simulink model "motor_dc_machine_block"  (R2025a)
settings: Solver=VariableStepAuto  StartTime=0.0  StopTime=2  RelTol=1e-3
undefined symbols (not defined in the file): J_m, kfi, L_a, R_a, T_n, V_an
libraries: spsControlledVoltageSourceLib x1, spsDCMachineLib x1, sps_lib x1
settings Model: Creator=SCH 2  LastModifiedBy=SCH 2

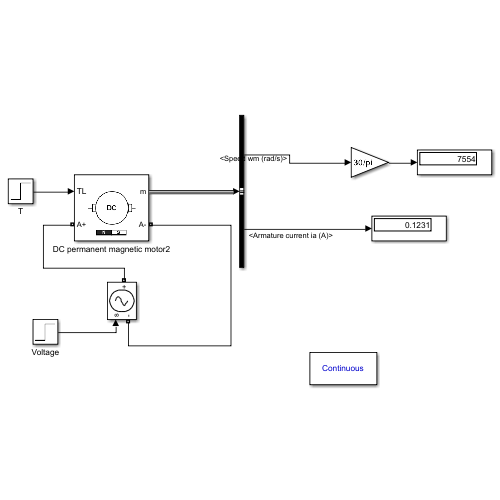
[thumbnail: Simulink's stored preview of the top-level diagram]
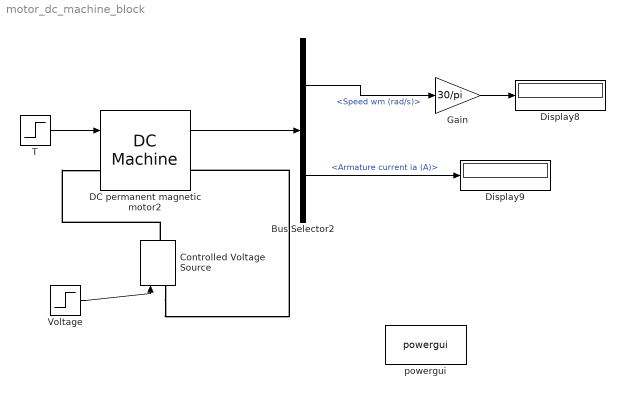
== system motor_dc_machine_block ==
  Bus Selector2 : BusSelector  OutputSignals=Speed wm (rad/s),Armature current ia (A)
  Controlled Voltage Source : spsControlledVoltageSourceLib/Controlled Voltage Source  Initialize=on  Source_Type=AC  Amplitude=0  Phase=0  Frequency=0  Measurements=None
  DC permanent magnetic motor2 : spsDCMachineLib/DC Machine  PresetModel=No  MechanicalLoad=Torque TL  FieldType=Permanent magnet  ShowDetailedParameters=on  MeasurementBus=off  RLa=[R_a L_a]  RLf=[180 71.47]  Laf=1.345  MachineConstant=Torque constant (N.m/A)  Ke=1.8  Kt=kfi  J=J_m  Bm=B_m  Tf=0  w0=1340.413  Ifinit=1  TsPowergui=0  TsBlock=-1
  Display8 : Display
  Display9 : Display
  Gain : Gain  Gain=30/pi
  T : Step  Time=2  After=T_n  SampleTime=0
  Voltage : Step  After=V_an  SampleTime=0
  powergui : sps_lib/powergui  Priority=1  SimulationMode=Continuous  SampleTime=50e-6  frequency=60  Iterations=50  frequencyindice=0  Pbase=100e6  ErrMax=1e-4  UnitsV=kV  UnitsW=MW  buscounter=0  FunctionMessages=off  echomessages=off  EnableUseOfTLC=off  CurrentSourceSwitches=off  DisableSnubberDevices=off  DisableRonSwitches=off  DisableVfSwitches=off  DisplayEquations=off  AutomaticDiscreteSolvers=off  SolverType=Tustin/Backward Euler (TBE)  Interpol=off  ExternalGateDelay=off  methode=off  Ts=100  x0status=blocks  SPID=on  SwTol=0  HookPort=off  NonlinearTolerance=1e-4  nMaxIteration=100  ContinueOnMaxIteration=off  RestoreLinks=warning  ResistiveCurrentMeasurement=off  Frange=[0:2:500]  Ylog=off  Xlog=on  ShowGrid=off  save=off  variable=ZData  structure=0  ZoomFFT=off  StartTime=0.0  cycles=1  DisplayStyle=1  fundamental=60  FreqAxis=off  MaxFrequency=1000  frequencyindicesteady=1  RmsSteady=1  display=off
  wires:
  Voltage/1 -> Controlled Voltage Source/1
  T/1 -> DC permanent magnetic motor2/1
  DC permanent magnetic motor2/1 -> Bus Selector2/1
  Bus Selector2/2 -> Display9/1  "<Armature current ia (A)>"
  Bus Selector2/1 -> Gain/1  "<Speed wm (rad/s)>"
  Gain/1 -> Display8/1
  connections:
  Controlled Voltage Source/RConn1 -- DC permanent magnetic motor2/LConn1
  Controlled Voltage Source/LConn1 -- DC permanent magnetic motor2/RConn1
